simulink library "lib_AC_SC"  (R2026a)
settings: Solver=VariableStepAuto
undefined symbols (not defined in the file): block_buses, block_idx, buses_lf, fref, Lbiginv, Nbuses, op_SC, SCs_buses
settings Model: Creator=atomas  LastModifiedBy=atomas

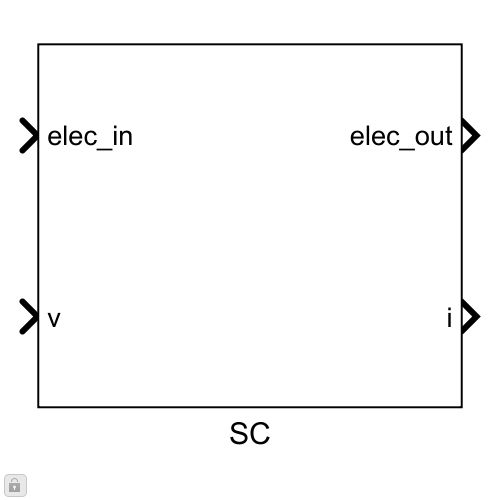
[thumbnail: Simulink's stored preview of the top-level diagram]
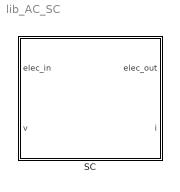
== system lib_AC_SC ==
  SC : Subsystem  mask(Synchronous machine){SCs_nodes=1, FBASE=50, D=0, H=8, Psimag_pu=0.8, Lssd_pu=1.6, Lssq_pu=0.66, Rs_pu=0.0018, Lmd_pu=1.5, Lmq_pu=0.56, Rfd_pu=0.00052277, Lfd_pu=0.14234, Rkd1_pu=0.0168, Lkd1_pu=0.08125, Rkd2_pu=10e6, Lkd2_pu=10e6, Rkq1_pu=10e6, Lkq1_pu=10e6, Rkq2_pu=10e6, Lkq2_pu=10e6, Rkq3_pu=10e6, Lkq3_pu=10e6, T_e=1.15, T_1=12, T_2=1, T_A=0.01, K_A=200, R_p=0.05, T_W=2, R_t=0.43, T_g=0.5, T_R=9}
      mask prompts: FBASE "Base frequency (Hz)"; D "Damping (pu)"; H "Inertia (s)"; Psimag_pu "Permanent flux (pu)"; Lssd_pu "Stator inductances (pu) Ld"; Lssq_pu "Stator inductances (pu) Lq"; Rs_pu "Stator resistances (pu)"; Lmd_pu "d-axis mutual inductance (pu)"; Lmq_pu "q-axis mutual inductance (pu)"; Rfd_pu "Excitation resistance (pu)"; Lfd_pu "Excitation inductance (pu)"; Rkd1_pu "d-axis damper resistance 1 (pu)"; Lkd1_pu "d-axis damper inductance 1 (pu)"; Rkd2_pu "d-axis damper resistance 2 (pu)"; Lkd2_pu "d-axis damper inductance 2 (pu)"; Rkq1_pu "q-axis damper resistance 1 (pu)"; Lkq1_pu "q-axis damper inductance 1 (pu)"; Rkq2_pu "q-axis damper resistance 2 (pu)"; Lkq2_pu "q-axis damper inductance 2 (pu)"; Rkq3_pu "q-axis damper resistance 3 (pu)"; Lkq3_pu "q-axis damper inductance 3 (pu)"
      mask help: Synchronous machine modelled in d-q reference frame.
      mask init:
      | [block_buses, block_idx, block_toM, block_fref, Lbiginv, Lssd_pu, Lssq_pu, Lmd_pu, Lmq_pu, Lfd_pu, Lkd1_pu, Lkd2_pu, Lkq1_pu, Lkq2_pu, Lkq3_pu] = mask_init_SC(gcb, Lssd_pu, Lssq_pu, Lmd_pu, Lmq_pu, Lfd_pu, Lkd1_pu, Lkd2_pu, Lkq1_pu, Lkq2_pu, Lkq3_pu);
      mask Help: web([extractBefore(get_param(bdroot, 'filename'),gcs) 'Documentation/SM.html'])
      mask DialogControl Params Prompt: Parameters
      mask DialogControl AVR Prompt: AVR
      mask DialogControl Gov Prompt: Speed governor

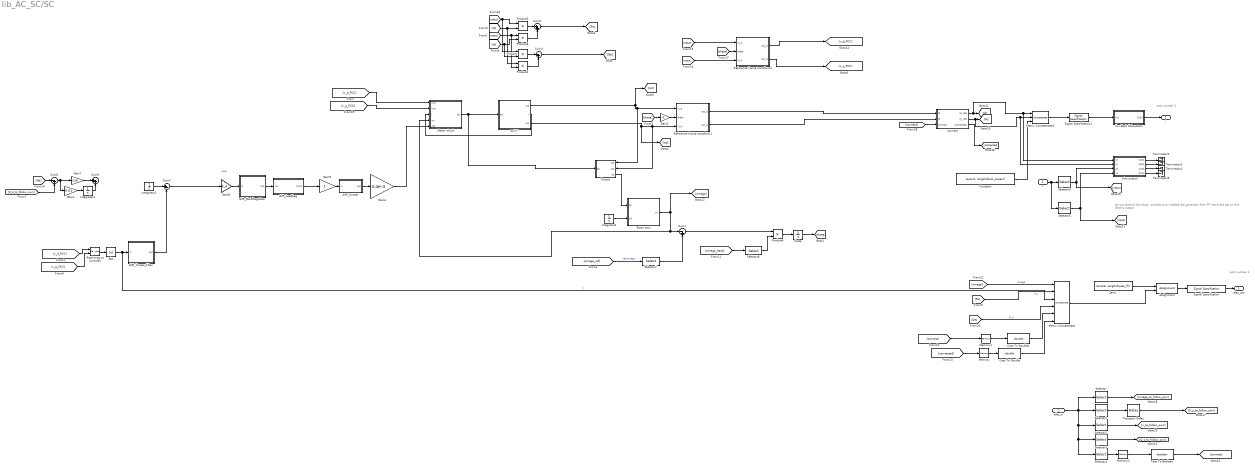
== system lib_AC_SC/SC ==
  note: AVR
  note: do not rename this block, conditions to initialise the generator from PF result are set on this block's output
  note: port number 1
  note: port number 2
  elec_in : Inport
  v : Inport  Port=2
  AVR_Exciter : Subsystem  mask{T_s=T_e}
      mask prompts: T_s "Filter time constant"
      mask Display:
      | try
      |     dpoly(1, [T_s, 1])
      | catch
      | end
  AVR_LeadLag : Subsystem  mask{T_2=T_2, T_1=T_1}
      mask help:
      | Transfer function:
      |
      |   1 + sT_2
      | ---------------
      |   1 + sT_1
      mask Display:
      | try
      |     dpoly([T_2, 1], [T_1, 1])
      | catch
      | end
  AVR_MainRegulator : Subsystem  mask{T_s=T_A}
      mask prompts: T_s "Filter time constant"
      mask Display:
      | try
      |     dpoly(1, [T_s, 1])
      | catch
      | end
  AVR_Vmeas_Filter : Subsystem  mask{T_r=0.01}
      mask prompts: T_r "Filter time constant"
      mask Display:
      | try
      |     dpoly(1, [T_r, 1])
      | catch
      | end
  Abs : Abs  SaturateOnIntegerOverflow=off
  Assignment : Assignment  NumberOfDimensions=2  DiagnosticForDimensions=Warning  IndexOptions=Assign all,Index vector (dialog)  Indices=1,block_idx  OutputSizes=1,1
  Cast To Boolean : DataTypeConversion  OutDataTypeStr=boolean  SaturateOnIntegerOverflow=off  RndMeth=Floor
  Cast To Double : DataTypeConversion  OutDataTypeStr=double  SaturateOnIntegerOverflow=off  RndMeth=Floor
  Cast To Double1 : DataTypeConversion  OutDataTypeStr=double  SaturateOnIntegerOverflow=off  RndMeth=Floor
  Constant : Constant  Value=zeros(1, length(block_buses))  VectorParams1D=off
  For Each Subsystem : Subsystem  TreatAsAtomicUnit=on
  Gain1 : Gain  Gain=0.01
  Gain2 : Gain  Gain=-1
  Gain4 : Gain  Gain=3.4e-4
  Gain7 : Gain  Gain=0.001
  Gain8 : Gain  Gain=K_A
  Gain9 : Gain
  Integrator1 : Integrator  InitialCondition=op_SC.Integrator1
  Integrator2 : Integrator  InitialCondition=op_SC.Integrator2
  Integrator3 : Integrator  InitialCondition=op_SC.Integrator3
  Matrix Concatenate : Concatenate  NumInputs=6  Mode=Multidimensional array
  Matrix Concatenate1 : Concatenate  NumInputs=3  Mode=Multidimensional array
  Memory : Memory  InitialCondition=1
  Memory1 : Memory  InitialCondition=1
  Memory2 : Memory  InitialCondition=1
  Product{,1..4} (5 alike) : Product
  Real-Imag to Complex : RealImagToComplex
  Reference frame transform1 : Subsystem
  Reference frame transform2 : Subsystem
  Rotor axis : Subsystem
  Selector : Selector  NumberOfDimensions=2  InputPortWidth=3  IndexOptions=Index vector (dialog),Index vector (dialog)  Indices=1,block_idx  OutputSizes=1,1
  Selector1 : Selector  NumberOfDimensions=2  InputPortWidth=3  IndexOptions=Index vector (dialog),Index vector (dialog)  Indices=2,block_idx  OutputSizes=1,1
  Selector2 : Selector  NumberOfDimensions=2  InputPortWidth=3  IndexOptions=Index vector (dialog),Index vector (dialog)  Indices=3,block_idx  OutputSizes=1,1
  Selector3 : Selector  NumberOfDimensions=2  InputPortWidth=3  IndexOptions=Index vector (dialog),Index vector (dialog)  Indices=4,block_idx  OutputSizes=1,1
  Selector4 : Selector  NumberOfDimensions=2  InputPortWidth=3  IndexOptions=Index vector (dialog),Index vector (dialog)  Indices=5,block_idx  OutputSizes=1,1
  Selector5 : Selector  NumberOfDimensions=2  InputPortWidth=3  IndexOptions=Index vector (dialog),Index vector (dialog)  Indices=1,block_buses  OutputSizes=1,1
  Selector6 : Selector  NumberOfDimensions=2  InputPortWidth=3  IndexOptions=Index vector (dialog),Index vector (dialog)  Indices=2,block_buses  OutputSizes=1,1
  Selector7 : Selector  InputPortWidth=length(fref.ref_units)  IndexOptions=Index vector (dialog)  Indices=block_fref  OutputSizes=1
  Selector8 : Selector  InputPortWidth=length(fref.ref_units)  IndexOptions=Index vector (dialog)  Indices=block_fref  OutputSizes=1
  Signal Specification : SignalSpecification  Dimensions=[6 length(buses_lf)]
  Signal Specification1 : SignalSpecification  Dimensions=[3 length(block_buses)]
  Stator circuit : Subsystem
  Sum1 : Sum  Inputs=|-+
  Sum2 : Sum  Inputs=|+-
  Sum4 : Sum  Inputs=|-+
  Sum5 : Sum  Inputs=|++
  Sum8 : Sum  Inputs=|-+
  Sum9 : Sum  Inputs=|++
  Terminator{2..5} (4 alike) : Terminator
  Torque : Subsystem
      settings: PortSchema="{\"entries\":[{\"content\":{\"sides\":[{\"content\":{\"connectorIds\":[\"In1\"]},\"type\":\"ConnectorPlacement.EquallySpacedRectSide\",\"uuid\":\"b7abd3bc-22dd-4669-aa40-98bc76884565\"},{\"content\":{\"connectorIds\":[\"In2\",\"In3\",\"Out1\"],\"side\":\"RIGHT\"},\"type\":\"ConnectorPlacement.EquallySpacedRectSide\",\"uuid\":\"e9abb552-b46d-48ed-aa1f-0e9dac604fea\"},{\"content\":{\"connectorIds\":[],\"side\":\"TOP\"},\"type\":\"ConnectorPlacement.EquallySpacedRectSide\",\"uuid\":\"4b14997d-8f32-4cfb-8a1b-18cffb093d28\"}]},\"type\":\"ConnectorPlacement.EquallySpacedConnector\",\"uuid\":\"d6624493-e930-4f0d-8cbe-17f96cb72edc\"}],\"packageUris\":[\"http://schema.mathworks.com/mf0/Connector/R2020b\"],\"version\":\"1.0\"}"
  Transport Delay : TransportDelay  DelayTime=0.0001  TransDelayFeedthrough=on
  Zero1 : Constant  Value=zeros(6, length(buses_lf))  VectorParams1D=off  OutDataTypeStr=Inherit: Inherit via back propagation
  connect : Subsystem
  psi->i : Subsystem
  theta : Integrator  InitialCondition=op_SC.theta  UpperSaturationLimit=2*pi  LowerSaturationLimit=0
  trim_output : Subsystem
  elec_out : Outport
  i : Outport  Port=2
  wires:
  Sum4/1 -> [Qe]
  Sum5/1 -> [Pe]
  [v_q_PCC] -> Real-Imag to Complex/2
  Real-Imag to Complex/1 -> Abs/1
  [v_d_PCC] -> Real-Imag to Complex/1
  [vqout] -> Product3/1, Product1/2
  [iq] -> Product3/2, Product/2
  Product/1 -> Sum4/1
  Product1/1 -> Sum4/2
  theta/1 -> [theta]
  psi->i/1(isd) -> Reference frame transform1/1(in_d), Torque/2(isd), [isd]
  psi->i/3(isq) -> [isq], Torque/3(isq), Reference frame transform1/3(in_q)
  Stator circuit/1(psi) -> Torque/1(psi), psi->i/1(psi)
  [v_q_PCC] -> Stator circuit/2(vsq)
  Gain2/1 -> Reference frame transform1/2(theta)
  Rotor axis/1(wr) -> Stator circuit/4(ws), Sum1/1, [omega]
  Torque/1(te) -> Rotor axis/1(te)
  [theta] -> Gain2/1
  psi->i/2(i) -> Stator circuit/3(i)
  [vdout] -> Product/1, Product2/1
  Product3/1 -> Sum5/2
  [omega_ref] -> Selector7/1  "ref_omega"
  Product2/1 -> Sum5/1
  [id] -> Product2/2, Product1/1
  [v_d_PCC] -> Stator circuit/1(vsd)
  Integrator2/1 -> Rotor axis/2(tm)
  Gain9/1 -> AVR_Exciter/1(in)
  AVR_Exciter/1(out) -> Gain4/1
  Sum2/1 -> Gain8/1
  AVR_LeadLag/1(Out1) -> Gain9/1
  Gain8/1 -> AVR_MainRegulator/1(in)
  AVR_MainRegulator/1(out) -> AVR_LeadLag/1(In1)
  Selector3/1 -> [Q_s_to_follow_own]
  Selector/1 -> [omega_to_follow_own]
  Selector2/1 -> [v_to_follow_own]
  Selector1/1 -> Transport Delay/1
  [Qe] -> Matrix Concatenate/4  "Q_s"
  [Pe] -> Matrix Concatenate/2  "P_s"
  Abs/1 -> Matrix Concatenate/3, AVR_Vmeas_Filter/1(in)  "v"
  [omega] -> Matrix Concatenate/1  "omega"
  Cast To Double/1 -> Matrix Concatenate/6
  [connected] -> Memory/1
  Cast To Double1/1 -> Matrix Concatenate/5
  [connect] -> Memory1/1
  [connect] -> connect/3(connect)
  connect/3(connected) -> [connected]
  connect/2(iq_real) -> Matrix Concatenate1/2, trim_output/2(iq), [iq]
  connect/1(id_real) -> Matrix Concatenate1/1, trim_output/1(id), [id]
  Cast To Boolean/1 -> [connect]
  Selector4/1 -> Memory2/1
  Sum8/1 -> Gain1/1, Gain7/1
  [Qe] -> Sum8/1
  Integrator3/1 -> Sum9/2
  Gain7/1 -> Sum9/1
  [Q_s_to_follow_own] -> Sum8/2
  Zero1/1 -> Assignment/1
  Signal Specification/1 -> elec_out/1
  elec_in/1 -> Selector4/1, Selector3/1, Selector2/1, Selector1/1, Selector/1
  Assignment/1 -> Signal Specification/1
  Matrix Concatenate/1 -> Assignment/2
  Matrix Concatenate1/1 -> Signal Specification1/1
  Signal Specification1/1 -> For Each Subsystem/1(In1)
  Constant/1 -> Matrix Concatenate1/3
  For Each Subsystem/1(Out1) -> i/1
  trim_output/1(Out1) -> Terminator2/1
  trim_output/2(Out2) -> Terminator3/1
  trim_output/4(Out4) -> Terminator5/1
  Selector5/1 -> trim_output/3(vd), [vdout]
  Selector6/1 -> [vqout], trim_output/4(vq)
  trim_output/3(Out3) -> Terminator4/1
  v/1 -> Selector6/1, Selector5/1
  Reference frame transform1/1(out_d) -> connect/1(id)
  Reference frame transform1/2(out_q) -> connect/2(iq)
  Gain1/1 -> Integrator3/1
  Memory/1 -> Cast To Double/1
  Memory1/1 -> Cast To Double1/1
  Memory2/1 -> Cast To Boolean/1
  Transport Delay/1 -> [P_s_to_follow_own]
  Reference frame transform2/1(out_d) -> [v_d_PCC]
  Reference frame transform2/2(out_q) -> [v_q_PCC]
  [theta] -> Reference frame transform2/2(theta)
  [vqout] -> Reference frame transform2/3(in_q)
  [vdout] -> Reference frame transform2/1(in_d)
  AVR_Vmeas_Filter/1(out) -> Sum2/2
  Gain4/1 -> Stator circuit/5(vfd)
  Integrator1/1 -> Sum2/1
  [omega_base] -> Selector8/1
  Selector8/1 -> Product4/2
  Product4/1 -> theta/1
  Sum1/1 -> Product4/1
  Selector7/1 -> Sum1/2

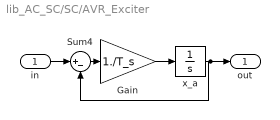
== system lib_AC_SC/SC/AVR_Exciter ==
  in : Inport
  Gain : Gain  Gain=1./T_s
  Sum4 : Sum  Inputs=|+-
  x_a : Integrator  InitialCondition=op_SC.AVR_Exciter_x_a
  out : Outport
  wires:
  Gain/1 -> x_a/1
  Sum4/1 -> Gain/1
  in/1 -> Sum4/1
  x_a/1 -> out/1, Sum4/2

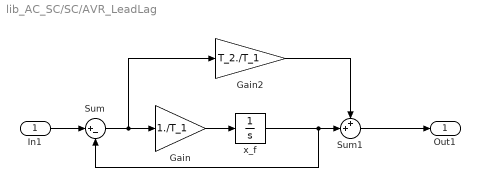
== system lib_AC_SC/SC/AVR_LeadLag ==
  In1 : Inport
  Gain : Gain  Gain=1./T_1
  Gain2 : Gain  Gain=T_2./T_1
  Sum : Sum  Inputs=|+-
  Sum1 : Sum  Inputs=++|
  x_f : Integrator  InitialCondition=op_SC.AVR_LeadLag_x_f
  Out1 : Outport
  wires:
  x_f/1 -> Sum1/2, Sum/2
  Gain/1 -> x_f/1
  Sum/1 -> Gain/1, Gain2/1
  Gain2/1 -> Sum1/1
  Sum1/1 -> Out1/1
  In1/1 -> Sum/1

== system lib_AC_SC/SC/AVR_MainRegulator ==
  in : Inport
  Gain : Gain  Gain=1./T_s
  Sum4 : Sum  Inputs=|+-
  x_a : Integrator  InitialCondition=op_SC.AVR_MainRegulator_x_a
  out : Outport
  wires:
  in/1 -> Sum4/1
  x_a/1 -> Sum4/2, out/1
  Sum4/1 -> Gain/1
  Gain/1 -> x_a/1

== system lib_AC_SC/SC/AVR_Vmeas_Filter ==
  in : Inport
  Gain : Gain  Gain=1./T_r
  Sum4 : Sum  Inputs=|+-
  x_a : Integrator  InitialCondition=op_SC.AVR_Vmeas_Filter_x_a
  out : Outport
  wires:
  Gain/1 -> x_a/1
  Sum4/1 -> Gain/1
  in/1 -> Sum4/1
  x_a/1 -> out/1, Sum4/2

== system lib_AC_SC/SC/For Each Subsystem ==
  In1 : Inport  Partition=on  PartitionDimension=1  PartitionWidth=1  PartitionOffset=0
  For Each : ForEach  DisableCoverage=on
  Gen_To : MATLAB Function  TreatAsAtomicUnit=on
  Out1 : Outport  ConcatenationDimension=1
  wires:
  Gen_To/1(y) -> Out1/1
  In1/1 -> Gen_To/1(u)

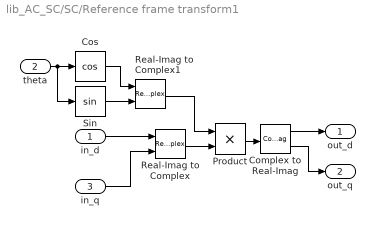
== system lib_AC_SC/SC/Reference frame transform1 ==
  in_d : Inport
  theta : Inport  Port=2
  in_q : Inport  Port=3
  Complex to Real-Imag : ComplexToRealImag
  Cos : Trigonometry  SCDEnableBlockLinearizationSpecification=on  Operator=cos
  Product : Product
  Real-Imag to Complex : RealImagToComplex
  Real-Imag to Complex1 : RealImagToComplex
  Sin : Trigonometry  SCDEnableBlockLinearizationSpecification=on
  out_d : Outport
  out_q : Outport  Port=2
  wires:
  in_d/1 -> Real-Imag to Complex/1
  in_q/1 -> Real-Imag to Complex/2
  Complex to Real-Imag/1 -> out_d/1
  Sin/1 -> Real-Imag to Complex1/2
  Cos/1 -> Real-Imag to Complex1/1
  theta/1 -> Cos/1, Sin/1
  Product/1 -> Complex to Real-Imag/1
  Real-Imag to Complex/1 -> Product/2
  Real-Imag to Complex1/1 -> Product/1
  Complex to Real-Imag/2 -> out_q/1

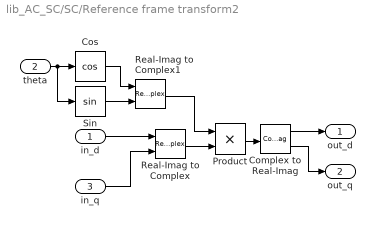
== system lib_AC_SC/SC/Reference frame transform2 ==
  in_d : Inport
  theta : Inport  Port=2
  in_q : Inport  Port=3
  Complex to Real-Imag : ComplexToRealImag
  Cos : Trigonometry  SCDEnableBlockLinearizationSpecification=on  Operator=cos
  Product : Product
  Real-Imag to Complex : RealImagToComplex
  Real-Imag to Complex1 : RealImagToComplex
  Sin : Trigonometry  SCDEnableBlockLinearizationSpecification=on
  out_d : Outport
  out_q : Outport  Port=2
  wires:
  in_d/1 -> Real-Imag to Complex/1
  in_q/1 -> Real-Imag to Complex/2
  Complex to Real-Imag/1 -> out_d/1
  Sin/1 -> Real-Imag to Complex1/2
  Cos/1 -> Real-Imag to Complex1/1
  theta/1 -> Cos/1, Sin/1
  Product/1 -> Complex to Real-Imag/1
  Real-Imag to Complex/1 -> Product/2
  Real-Imag to Complex1/1 -> Product/1
  Complex to Real-Imag/2 -> out_q/1

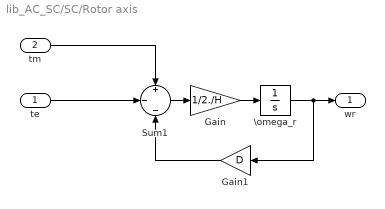
== system lib_AC_SC/SC/Rotor axis ==
  te : Inport
  tm : Inport  Port=2
  Gain : Gain  Gain=1/2./H
  Gain1 : Gain  Gain=D
  Sum1 : Sum  Inputs=+|-|-  InputSameDT=on  SaturateOnIntegerOverflow=on  OutDataTypeStr=Inherit: Same as first input
  \omega_r : Integrator  InitialCondition=op_SC.Rotor_axis_omega_r  UpperSaturationLimit=2*pi  LowerSaturationLimit=0
  wr : Outport  VectorParamsAs1DForOutWhenUnconnected=off
  wires:
  tm/1 -> Sum1/1
  \omega_r/1 -> wr/1, Gain1/1
  te/1 -> Sum1/2
  Sum1/1 -> Gain/1
  Gain/1 -> \omega_r/1
  Gain1/1 -> Sum1/3

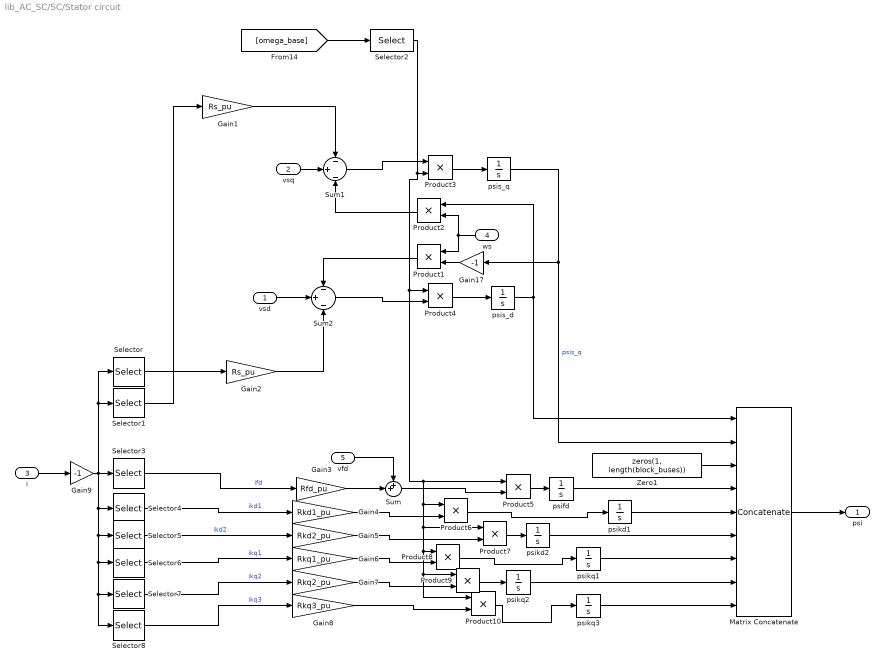
== system lib_AC_SC/SC/Stator circuit ==
  vsd : Inport
  vsq : Inport  Port=2
  i : Inport  Port=3
  ws : Inport  Port=4
  vfd : Inport  Port=5
  Gain1 : Gain  Gain=Rs_pu
  Gain17 : Gain  Gain=-1
  Gain2 : Gain  Gain=Rs_pu
  Gain3 : Gain  Gain=Rfd_pu
  Gain4 : Gain  Gain=Rkd1_pu
  Gain5 : Gain  Gain=Rkd2_pu
  Gain6 : Gain  Gain=Rkq1_pu
  Gain7 : Gain  Gain=Rkq2_pu
  Gain8 : Gain  Gain=Rkq3_pu
  Gain9 : Gain  Gain=-1
  Matrix Concatenate : Concatenate  NumInputs=9  Mode=Multidimensional array
  Product{1..10} (10 alike) : Product
  Selector : Selector  NumberOfDimensions=2  InputPortWidth=9  IndexOptions=Index vector (dialog),Select all  Indices=[1],1  OutputSizes=1,1
  Selector1 : Selector  NumberOfDimensions=2  InputPortWidth=9  IndexOptions=Index vector (dialog),Select all  Indices=[2],1  OutputSizes=1,1
  Selector2 : Selector  InputPortWidth=length(fref.ref_units)  IndexOptions=Index vector (dialog)  Indices=block_fref  OutputSizes=1
  Selector3 : Selector  NumberOfDimensions=2  InputPortWidth=9  IndexOptions=Index vector (dialog),Select all  Indices=[4],1  OutputSizes=1,1
  Selector4 : Selector  NumberOfDimensions=2  InputPortWidth=9  IndexOptions=Index vector (dialog),Select all  Indices=[5],1  OutputSizes=1,1
  Selector5 : Selector  NumberOfDimensions=2  InputPortWidth=9  IndexOptions=Index vector (dialog),Select all  Indices=[6],1  OutputSizes=1,1
  Selector6 : Selector  NumberOfDimensions=2  InputPortWidth=9  IndexOptions=Index vector (dialog),Select all  Indices=[7],1  OutputSizes=1,1
  Selector7 : Selector  NumberOfDimensions=2  InputPortWidth=9  IndexOptions=Index vector (dialog),Select all  Indices=[8],1  OutputSizes=1,1
  Selector8 : Selector  NumberOfDimensions=2  InputPortWidth=9  IndexOptions=Index vector (dialog),Select all  Indices=[9],1  OutputSizes=1,1
  Sum : Sum  Inputs=++|
  Sum1 : Sum  Inputs=-|+|-  InputSameDT=on  SaturateOnIntegerOverflow=on  OutDataTypeStr=Inherit: Same as first input
  Sum2 : Sum  Inputs=-|+|-  InputSameDT=on  SaturateOnIntegerOverflow=on  OutDataTypeStr=Inherit: Same as first input
  Zero1 : Constant  Value=zeros(1, length(block_buses))  VectorParams1D=off  OutDataTypeStr=Inherit: Inherit via back propagation
  psifd : Integrator  InitialCondition=op_SC.Stator_circuit_psifd
  psikd1 : Integrator  InitialCondition=op_SC.Stator_circuit_psikd1
  psikd2 : Integrator  InitialCondition=op_SC.Stator_circuit_psikd2
  psikq1 : Integrator  InitialCondition=op_SC.Stator_circuit_psikq1
  psikq2 : Integrator  InitialCondition=op_SC.Stator_circuit_psikq2
  psikq3 : Integrator  InitialCondition=op_SC.Stator_circuit_psikq3
  psis_d : Integrator  InitialCondition=op_SC.Stator_circuit_psis_d
  psis_q : Integrator  InitialCondition=op_SC.Stator_circuit_psis_q
  psi : Outport  VectorParamsAs1DForOutWhenUnconnected=off
  wires:
  Product3/1 -> psis_q/1
  Sum1/1 -> Product3/1
  Selector3/1 -> Gain3/1  "ifd"
  Selector8/1 -> Gain8/1  "ikq3"
  Selector7/1 -> Gain7/1  "ikq2"
  Selector6/1 -> Gain6/1  "ikq1"
  Selector5/1 -> Gain5/1  "ikd2"
  Selector4/1 -> Gain4/1  "ikd1"
  Gain3/1 -> Sum/2
  vfd/1 -> Sum/1
  Sum/1 -> Product5/2
  Gain4/1 -> Product6/2
  Gain6/1 -> Product8/2
  Gain8/1 -> Product10/2
  Gain7/1 -> Product9/2
  psikd2/1 -> Matrix Concatenate/6
  psifd/1 -> Matrix Concatenate/4
  psikq3/1 -> Matrix Concatenate/9
  psikq1/1 -> Matrix Concatenate/7
  psikd1/1 -> Matrix Concatenate/5
  Matrix Concatenate/1 -> psi/1
  i/1 -> Gain9/1
  Product5/1 -> psifd/1
  Product6/1 -> psikd1/1
  Product7/1 -> psikd2/1
  Product8/1 -> psikq1/1
  Product9/1 -> psikq2/1
  Product10/1 -> psikq3/1
  Gain9/1 -> Selector8/1, Selector7/1, Selector6/1, Selector5/1, Selector4/1, Selector1/1, Selector/1, Selector3/1
  psikq2/1 -> Matrix Concatenate/8
  Zero1/1 -> Matrix Concatenate/3
  vsd/1 -> Sum2/2
  Sum2/1 -> Product4/2
  Product4/1 -> psis_d/1
  ws/1 -> Product1/1, Product2/2
  Gain17/1 -> Product1/2
  psis_q/1 -> Matrix Concatenate/2, Gain17/1  "psis_q"
  Product1/1 -> Sum2/1
  Product2/1 -> Sum1/3
  psis_d/1 -> Product2/1, Matrix Concatenate/1
  Selector/1 -> Gain2/1
  Gain2/1 -> Sum2/3
  Selector1/1 -> Gain1/1
  Gain1/1 -> Sum1/1
  vsq/1 -> Sum1/2
  [omega_base] -> Selector2/1
  Selector2/1 -> Product10/1, Product9/1, Product8/1, Product7/1, Product6/1, Product5/1, Product4/1, Product3/2
  Gain5/1 -> Product7/2

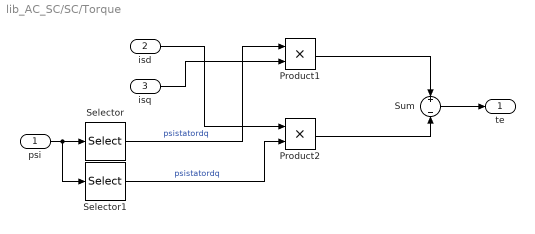
== system lib_AC_SC/SC/Torque ==
  psi : Inport
  isd : Inport  Port=2
  isq : Inport  Port=3
  Product1 : Product
  Product2 : Product
  Selector : Selector  NumberOfDimensions=2  InputPortWidth=9  IndexOptions=Index vector (dialog),Select all  Indices=[1],1  OutputSizes=1,1
  Selector1 : Selector  NumberOfDimensions=2  InputPortWidth=9  IndexOptions=Index vector (dialog),Select all  Indices=[2],1  OutputSizes=1,1
  Sum : Sum  Inputs=+||-
  te : Outport  VectorParamsAs1DForOutWhenUnconnected=off
  wires:
  Product1/1 -> Sum/1
  Sum/1 -> te/1
  Selector/1 -> Product1/1  "psistatordq"
  psi/1 -> Selector1/1, Selector/1
  Product2/1 -> Sum/2
  isq/1 -> Product1/2
  isd/1 -> Product2/1
  Selector1/1 -> Product2/2  "psistatordq"

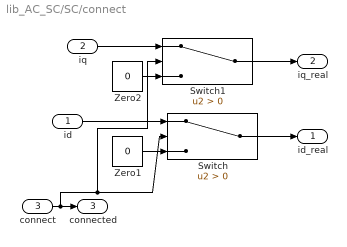
== system lib_AC_SC/SC/connect ==
  id : Inport
  iq : Inport  Port=2
  connect : Inport  Port=3
  Switch : Switch  Criteria=u2 > Threshold  ZeroCross=off  SaturateOnIntegerOverflow=off  InputSameDT=off
  Switch1 : Switch  Criteria=u2 > Threshold  ZeroCross=off  SaturateOnIntegerOverflow=off  InputSameDT=off
  Zero1 : Constant  Value=0  VectorParams1D=off  OutDataTypeStr=Inherit: Inherit via back propagation
  Zero2 : Constant  Value=0  VectorParams1D=off  OutDataTypeStr=Inherit: Inherit via back propagation
  id_real : Outport
  iq_real : Outport  Port=2
  connected : Outport  Port=3  OutDataTypeStr=boolean
  wires:
  Switch/1 -> id_real/1
  Zero1/1 -> Switch/3
  id/1 -> Switch/1
  connect/1 -> connected/1, Switch1/2, Switch/2
  Switch1/1 -> iq_real/1
  iq/1 -> Switch1/1
  Zero2/1 -> Switch1/3

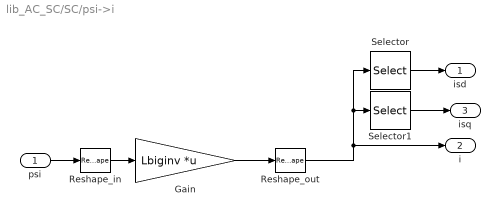
== system lib_AC_SC/SC/psi->i ==
  psi : Inport
  Gain : Gain  Gain=Lbiginv  Multiplication=Matrix(K*u)
  Reshape_in : Reshape  OutputDimensionality=Column vector (2-D)
  Reshape_out : Reshape  OutputDimensionality=Customize  OutputDimensions=[9, length(SCs_buses)]
  Selector : Selector  NumberOfDimensions=2  InputPortWidth=9  IndexOptions=Index vector (dialog),Select all  Indices=[1],1  OutputSizes=1,1
  Selector1 : Selector  NumberOfDimensions=2  InputPortWidth=9  IndexOptions=Index vector (dialog),Select all  Indices=[2],1  OutputSizes=1,1
  isd : Outport  VectorParamsAs1DForOutWhenUnconnected=off
  i : Outport  Port=2  VectorParamsAs1DForOutWhenUnconnected=off
  isq : Outport  Port=3  VectorParamsAs1DForOutWhenUnconnected=off
  wires:
  Selector/1 -> isd/1
  Gain/1 -> Reshape_out/1
  psi/1 -> Reshape_in/1
  Reshape_in/1 -> Gain/1
  Reshape_out/1 -> Selector1/1, Selector/1, i/1
  Selector1/1 -> isq/1

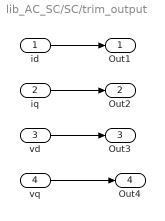
== system lib_AC_SC/SC/trim_output ==
  id : Inport
  iq : Inport  Port=2
  vd : Inport  Port=3
  vq : Inport  Port=4
  Out1 : Outport
  Out2 : Outport  Port=2
  Out3 : Outport  Port=3
  Out4 : Outport  Port=4
  wires:
  id/1 -> Out1/1
  vq/1 -> Out4/1
  vd/1 -> Out3/1
  iq/1 -> Out2/1

== matlab function lib_AC_SC/SC/For Each Subsystem/Gen_To ==
  data: u input; y output; Nbuses parameter; block_buses parameter
function y = fcn(u, Nbuses, block_buses)

y = zeros(1, Nbuses);
for i=1:Nbuses
    y(i) = sum(u(block_buses == i));
end
